simulink model "LAB1simulink"  (R2026b)
settings: Solver=VariableStepAuto
values from neighbouring files (symbols this model uses):
  cpp = 1000    [LAB1.m]
  Cv1 = cpp * rop * Vp1    (= 108000)    [LAB1.m]
  Cv2 = cpp * rop * Vp2    (= 72000)    [LAB1.m]
  czas_skok = 100    [LAB1.m]
  dFp = wart_skok2(skok,2)    [LAB1.m]
  dTkz = wart_skok2(skok,1)    [LAB1.m]
  dTzew = wart_skok2(skok,3)    [LAB1.m]
  Fp0 = punkt_pracy2(punkt,3)    [LAB1.m]
  K0 = (PkN - Ks1 * (Tw1N - TzewN))/(Tw1N-Tw2N)    (= 608.695652174)    [LAB1.m]
  Ks1 = a*Ks2    (= 173.913043478)    [LAB1.m]
  Ks2 = PkN/(a*(Tw1N - TzewN) + (Tw2N - TzewN))    (= 86.9565217391)    [LAB1.m]
  rop = 1.2    [LAB1.m]
  Tkz0 = punkt_pracy2(punkt,2)    [LAB1.m]
  Tw10 = (cpp*rop*Fp0*Tkz0 + Ks1*Tzew0 + K0*(Ks2*Tzew0)/(Ks2+K0)) / (cpp*rop*Fp0 + Ks1 + K0 - K0^2/(Ks2+K0))    (= 20)    [LAB1.m]
  Tw20 = (K0*Tw10 + Ks2*Tzew0)/(Ks2+K0)    (= 15)    [LAB1.m]
  Tzew0 = punkt_pracy2(punkt,1)    [LAB1.m]
settings Model: Creator=janhulboj  LastModifiedBy=janhulboj

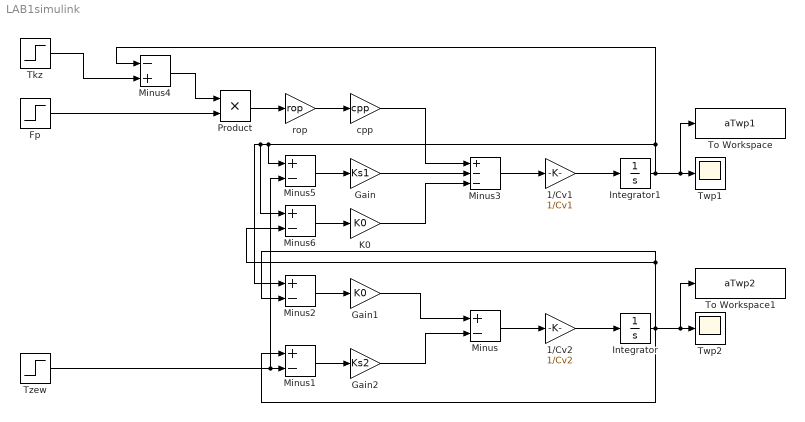
== system LAB1simulink ==
  1/Cv1 : Gain  Gain=1/Cv1
  1/Cv2 : Gain  Gain=1/Cv2
  Fp : Step  Time=czas_skok  InitialValue=Fp0  FinalValue=Fp0 + dFp  SampleTime=0
  Gain : Gain  Gain=Ks1
  Gain1 : Gain  Gain=K0
  Gain2 : Gain  Gain=Ks2
  Integrator : Integrator  InitialCondition=Tw20
  Integrator1 : Integrator  InitialCondition=Tw10
  K0 : Gain  Gain=K0
  Minus{,1..2,5..6} (5 alike) : Sum  Inputs=+-
  Minus3 : Sum  Inputs=+--
  Minus4 : Sum  Inputs=-+
  Product : Product
  Tkz : Step  Time=czas_skok  InitialValue=Tkz0  FinalValue=Tkz0 + dTkz  SampleTime=0
  To Workspace : ToWorkspace  VariableName=aTwp1  SampleTime=-1
      settings: Save2DSignal=2-D array (concatenate along first dimension)
  To Workspace1 : ToWorkspace  VariableName=aTwp2  SampleTime=-1
      settings: Save2DSignal=2-D array (concatenate along first dimension)
  Twp1 : Scope
      settings: ActiveDisplayYMinimum=-32.641902963192877  ActiveDisplayYMaximum=69.2472396777806
  Twp2 : Scope
      settings: ActiveDisplayYMinimum=14.846769695849733  ActiveDisplayYMaximum=16.379072737352406
  Tzew : Step  Time=czas_skok  InitialValue=Tzew0  FinalValue=Tzew0 + dTzew  SampleTime=0
  cpp : Gain  Gain=cpp
  rop : Gain  Gain=rop
  wires:
  Integrator/1 -> Minus6/2, Minus2/2, To Workspace1/1, Twp2/1, Minus1/1
  1/Cv2/1 -> Integrator/1
  Minus/1 -> 1/Cv2/1
  Gain1/1 -> Minus/1
  Gain2/1 -> Minus/2
  Minus2/1 -> Gain1/1
  Minus1/1 -> Gain2/1
  Tzew/1 -> Minus5/2, Minus1/2
  Integrator1/1 -> Minus2/1, Minus6/1, Minus5/1, Minus4/1, To Workspace/1, Twp1/1
  1/Cv1/1 -> Integrator1/1
  Minus3/1 -> 1/Cv1/1
  cpp/1 -> Minus3/1
  rop/1 -> cpp/1
  Product/1 -> rop/1
  Minus4/1 -> Product/1
  Tkz/1 -> Minus4/2
  Fp/1 -> Product/2
  Gain/1 -> Minus3/2
  K0/1 -> Minus3/3
  Minus5/1 -> Gain/1
  Minus6/1 -> K0/1
